simulink model "PSO_BON"  (R2019b)
settings: Solver=VariableStepAuto  StartTime=0.0  StopTime=0.2  RelTol=1e-5
undefined symbols (not defined in the file): sigbuilder_block
libraries: powerlib x164, re_lib x96, powerlib_meascontrol x9
(part 1 of 6)
settings Model: Creator=Mahesh Krishna  LastModifiedBy=nanaud
settings SolverCC: MaxConsecutiveZCs=1000000  AlgebraicLoopSolver=LineSearch  AutoInsertRateTranBlk=on
settings DataIOCC: ReturnWorkspaceOutputs=off
settings OptimizationCC: LifeSpan=inf
settings DebuggingCC: IgnoredZcDiagnostic=none  ArithmeticOperatorsInVariantConditions=warning
settings SFSimCC: SimUseLocalCustomCode=off  CustomCodeUndefinedFunction=UseInterfaceOnly
settings RTWCC: RTWUseLocalCustomCode=off
settings CodeAppCC: StateflowObjectComments=on
settings SimscapeCC: SimscapeNormalizeSystem=off

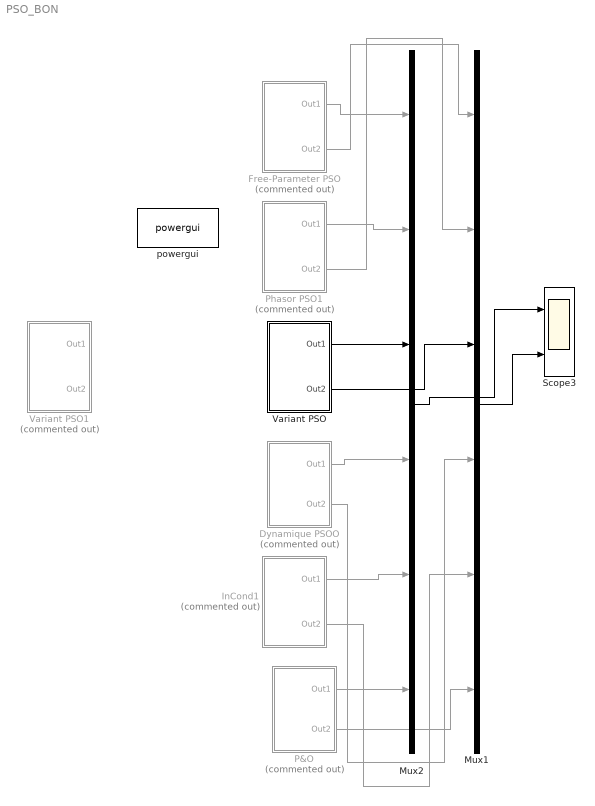
== system PSO_BON ==
  Dynamique PSOO : Subsystem  Commented=on
  Free-Parameter PSO : Subsystem  Commented=on
  InCond1 : Subsystem  Commented=on
  Mux1 : Mux  Inputs=6
  Mux2 : Mux  Inputs=6
  P&O : Subsystem  Commented=on
  Phasor PSO1 : Subsystem  Commented=on
  Scope3 : Scope  NumInputPorts=2
  Variant PSO : Subsystem
  Variant PSO1 : Subsystem  Commented=on
  powergui : powerlib/powergui  Priority=1  SimulationMode=Continuous  SampleTime=1e-6  frequency=60  Iterations=50  frequencyindice=0  Pbase=100e6  ErrMax=1e-4  UnitsV=kV  UnitsW=MW  buscounter=0  FunctionMessages=off  echomessages=off  EnableUseOfTLC=off  CurrentSourceSwitches=off  DisableSnubberDevices=off  DisableRonSwitches=off  DisableVfSwitches=off  DisplayEquations=off  AutomaticDiscreteSolvers=off  SolverType=Tustin/Backward Euler (TBE)  Interpol=off  ExternalGateDelay=off  methode=off  Ts=100  x0status=blocks  SPID=on  SwTol=0  HookPort=off  NonlinearTolerance=1e-4  nMaxIteration=100  ContinueOnMaxIteration=off  RestoreLinks=warning  ResistiveCurrentMeasurement=off  Frange=[0:2:500]  Ylog=off  Xlog=on  ShowGrid=off  save=off  variable=ZData  structure=0  ZoomFFT=off  StartTime=0.0  cycles=1  DisplayStyle=1  fundamental=60  FreqAxis=off  MaxFrequency=1000  frequencyindicesteady=1  RmsSteady=1  display=off
      settings: SourceProductName=Simscape Electrical
  wires:
  Mux2/1 -> Scope3/1
  Mux1/1 -> Scope3/2
  Free-Parameter PSO/1(Out1) -> Mux2/1
  P&O/1(Out1) -> Mux2/6
  InCond1/1(Out1) -> Mux2/5
  Dynamique PSOO/1(Out1) -> Mux2/4
  Variant PSO/1(Out1) -> Mux2/3
  Phasor PSO1/1(Out1) -> Mux2/2
  Free-Parameter PSO/2(Out2) -> Mux1/1
  Phasor PSO1/2(Out2) -> Mux1/2
  Variant PSO/2(Out2) -> Mux1/3
  Dynamique PSOO/2(Out2) -> Mux1/4
  InCond1/2(Out2) -> Mux1/5
  P&O/2(Out2) -> Mux1/6

== system PSO_BON/Dynamique PSOO ==
  Diode1 : powerlib/Power Electronics/Diode  Ron=1e-3  Lon=0  Vf=0  IC=0  UseSnubber=off  Rs=inf  Cs=inf  Measurements=off
      settings: SourceProductName=Simscape Electrical
  I : powerlib/Measurements/Current Measurement  PhasorSimulation=off  OutputType=Magnitude  PSBequivalent=0
      settings: SourceProductName=Simscape Electrical
  L : powerlib/Elements/Series RLC Branch  LConnTagsString=__new0  RConnTagsString=__new0  BranchType=L  Resistance=1e-3  Inductance=5e-3  SetiL0=off  InitialCurrent=0  Capacitance=1e-6  Setx0=off  InitialVoltage=0  Measurements=None
      settings: SourceProductName=Simscape Electrical
  M : powerlib/Power Electronics/Mosfet  Ron=1e-3  Lon=0  Rd=1e-3  Vfd=0  IC=0  Rs=inf  Cs=inf  Measurements=off
      settings: SourceProductName=Simscape Electrical
  MATLAB Function1 : MATLAB Function  TreatAsAtomicUnit=on
  Memory1 : Memory  LinearizeMemory=on
  Memory2 : Memory  LinearizeMemory=on
  Memory3 : Memory  LinearizeMemory=on
  PWM Generator (DC-DC)1 : powerlib_meascontrol/Pulse & Signal Generators/PWM Generator (DC-DC)  Fsw=40000  Ts=0
      settings: SourceProductName=Simscape Electrical
  Panel Surya : Subsystem
  Product1 : Product
  Saturation [0...1] : Saturate  UpperLimit=1  LowerLimit=0
  Series RLC Branch1 : powerlib/Elements/Series RLC Branch  LConnTagsString=__new0  RConnTagsString=__new0  BranchType=C  Resistance=1e-4  Inductance=200e-6  SetiL0=off  InitialCurrent=0  Capacitance=1e-6  Setx0=off  InitialVoltage=40  Measurements=None
      settings: SourceProductName=Simscape Electrical
  Series RLC Branch3 : powerlib/Elements/Series RLC Branch  LConnTagsString=__new0  RConnTagsString=__new0  BranchType=R  Resistance=100  Inductance=200e-6  SetiL0=off  InitialCurrent=0  Capacitance=1000e-6  Setx0=off  InitialVoltage=40  Measurements=None
      settings: SourceProductName=Simscape Electrical
  To Workspace4 : ToWorkspace  VariableName=Power5  SaveFormat=Structure With Time  SampleTime=-1
  To Workspace5 : ToWorkspace  VariableName=Duty5  SaveFormat=Structure With Time  SampleTime=-1
  Voltage Measurement1 : powerlib/Measurements/Voltage Measurement  PhasorSimulation=off  OutputType=Magnitude  PSBequivalent=0
      settings: SourceProductName=Simscape Electrical
  c : powerlib/Elements/Series RLC Branch  LConnTagsString=__new0  RConnTagsString=__new0  BranchType=C  Resistance=1e-3  Inductance=250e-6  SetiL0=off  InitialCurrent=0  Capacitance=10e-6  Setx0=off  InitialVoltage=0  Measurements=None
      settings: SourceProductName=Simscape Electrical
  Out1 : Outport
  Out2 : Outport  Port=2
  wires:
  Memory3/1 -> MATLAB Function1/2(Ipv)
  Memory2/1 -> MATLAB Function1/1(Vpv)
  I/1 -> [Ipv]
  Voltage Measurement1/1 -> [Vpv]
  PWM Generator (DC-DC)1/1 -> M/1
  Memory1/1 -> PWM Generator (DC-DC)1/1, To Workspace5/1, Out2/1
  Product1/1 -> To Workspace4/1, Out1/1
  [Ipv] -> Product1/1, Memory3/1
  [Vpv] -> Product1/2, Memory2/1
  MATLAB Function1/1(D) -> Saturation [0...1]/1
  Saturation [0...1]/1 -> Memory1/1
  connections:
  Panel Surya/RConn1 -- I/LConn1
  L/RConn1 -- M/LConn1 -- Diode1/LConn1
  Series RLC Branch1/LConn1 -- Diode1/RConn1 -- Series RLC Branch3/LConn1
  M/RConn1 -- Series RLC Branch3/RConn1 -- Series RLC Branch1/RConn1 -- c/RConn1 -- Panel Surya/RConn2 -- Voltage Measurement1/LConn2
  L/LConn1 -- c/LConn1 -- Voltage Measurement1/LConn1 -- I/RConn1

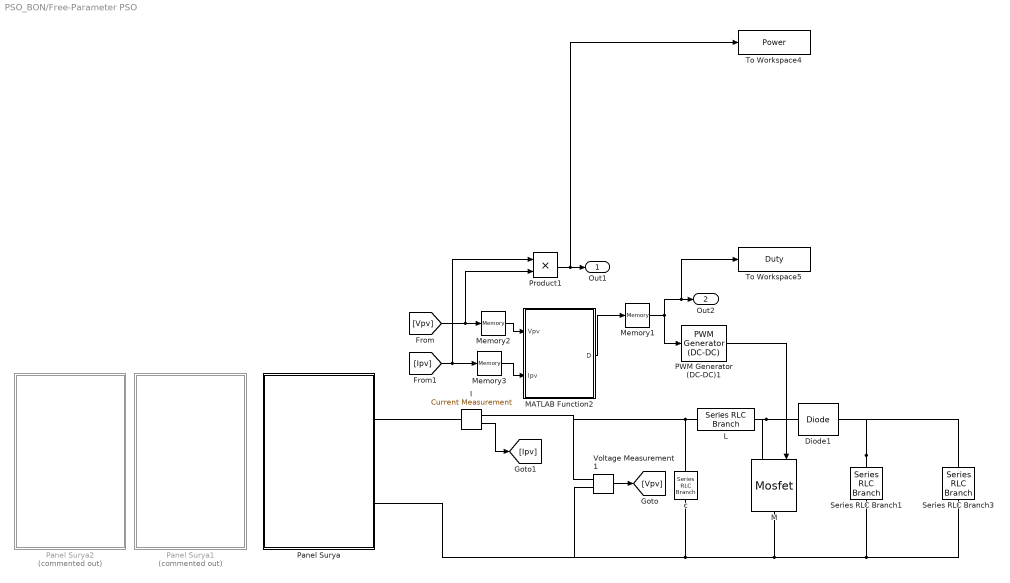
== system PSO_BON/Free-Parameter PSO ==
  Diode1 : powerlib/Power Electronics/Diode  Ron=1e-3  Lon=0  Vf=0  IC=0  UseSnubber=off  Rs=inf  Cs=inf  Measurements=off
      settings: SourceProductName=Simscape Electrical
  I : powerlib/Measurements/Current Measurement  PhasorSimulation=off  OutputType=Magnitude  PSBequivalent=0
      settings: SourceProductName=Simscape Electrical
  L : powerlib/Elements/Series RLC Branch  LConnTagsString=__new0  RConnTagsString=__new0  BranchType=L  Resistance=1e-3  Inductance=5e-3  SetiL0=off  InitialCurrent=0  Capacitance=1e-6  Setx0=off  InitialVoltage=0  Measurements=None
      settings: SourceProductName=Simscape Electrical
  M : powerlib/Power Electronics/Mosfet  Ron=1e-3  Lon=0  Rd=1e-3  Vfd=0  IC=0  Rs=inf  Cs=inf  Measurements=off
      settings: SourceProductName=Simscape Electrical
  MATLAB Function2 : MATLAB Function  TreatAsAtomicUnit=on
  Memory1 : Memory  LinearizeMemory=on
  Memory2 : Memory  LinearizeMemory=on
  Memory3 : Memory  LinearizeMemory=on
  PWM Generator (DC-DC)1 : powerlib_meascontrol/Pulse & Signal Generators/PWM Generator (DC-DC)  Fsw=40000  Ts=0
      settings: SourceProductName=Simscape Electrical
  Panel Surya : Subsystem
  Panel Surya1 : Subsystem  Commented=on
  Panel Surya2 : Subsystem  Commented=on
  Product1 : Product
  Series RLC Branch1 : powerlib/Elements/Series RLC Branch  LConnTagsString=__new0  RConnTagsString=__new0  BranchType=C  Resistance=1e-4  Inductance=200e-6  SetiL0=off  InitialCurrent=0  Capacitance=1e-6  Setx0=off  InitialVoltage=40  Measurements=None
      settings: SourceProductName=Simscape Electrical
  Series RLC Branch3 : powerlib/Elements/Series RLC Branch  LConnTagsString=__new0  RConnTagsString=__new0  BranchType=R  Resistance=100  Inductance=200e-6  SetiL0=off  InitialCurrent=0  Capacitance=1000e-6  Setx0=off  InitialVoltage=40  Measurements=None
      settings: SourceProductName=Simscape Electrical
  To Workspace4 : ToWorkspace  VariableName=Power  SaveFormat=Structure With Time  SampleTime=-1
  To Workspace5 : ToWorkspace  VariableName=Duty  SaveFormat=Structure With Time  SampleTime=-1
  Voltage Measurement1 : powerlib/Measurements/Voltage Measurement  PhasorSimulation=off  OutputType=Magnitude  PSBequivalent=0
      settings: SourceProductName=Simscape Electrical
  c : powerlib/Elements/Series RLC Branch  LConnTagsString=__new0  RConnTagsString=__new0  BranchType=C  Resistance=1e-3  Inductance=250e-6  SetiL0=off  InitialCurrent=0  Capacitance=10e-6  Setx0=off  InitialVoltage=0  Measurements=None
      settings: SourceProductName=Simscape Electrical
  Out1 : Outport
  Out2 : Outport  Port=2
  wires:
  Memory3/1 -> MATLAB Function2/2(Ipv)
  Memory2/1 -> MATLAB Function2/1(Vpv)
  I/1 -> [Ipv]
  Voltage Measurement1/1 -> [Vpv]
  PWM Generator (DC-DC)1/1 -> M/1
  Memory1/1 -> PWM Generator (DC-DC)1/1, To Workspace5/1, Out2/1
  Product1/1 -> To Workspace4/1, Out1/1
  [Ipv] -> Product1/1, Memory3/1
  MATLAB Function2/1(D) -> Memory1/1
  [Vpv] -> Product1/2, Memory2/1
  connections:
  Panel Surya/RConn1 -- I/LConn1
  L/RConn1 -- M/LConn1 -- Diode1/LConn1
  Series RLC Branch1/LConn1 -- Diode1/RConn1 -- Series RLC Branch3/LConn1
  M/RConn1 -- Series RLC Branch3/RConn1 -- Series RLC Branch1/RConn1 -- c/RConn1 -- Panel Surya/RConn2 -- Voltage Measurement1/LConn2
  L/LConn1 -- c/LConn1 -- Voltage Measurement1/LConn1 -- I/RConn1

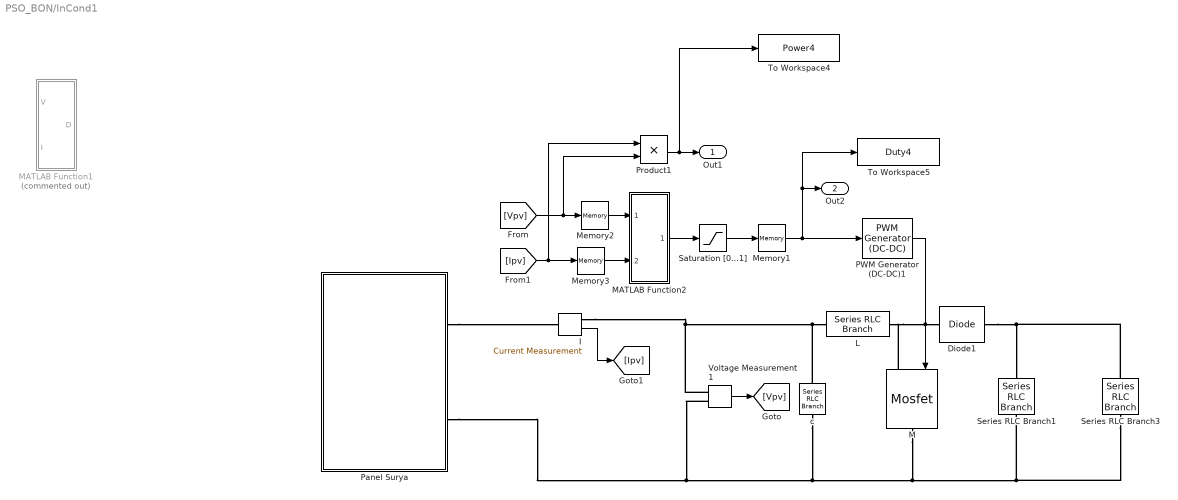
== system PSO_BON/InCond1 ==
  Diode1 : powerlib/Power Electronics/Diode  Ron=1e-3  Lon=0  Vf=0  IC=0  UseSnubber=off  Rs=inf  Cs=inf  Measurements=off
      settings: SourceProductName=Simscape Electrical
  I : powerlib/Measurements/Current Measurement  PhasorSimulation=off  OutputType=Magnitude  PSBequivalent=0
      settings: SourceProductName=Simscape Electrical
  L : powerlib/Elements/Series RLC Branch  LConnTagsString=__new0  RConnTagsString=__new0  BranchType=L  Resistance=1e-3  Inductance=5e-3  SetiL0=off  InitialCurrent=0  Capacitance=1e-6  Setx0=off  InitialVoltage=0  Measurements=None
      settings: SourceProductName=Simscape Electrical
  M : powerlib/Power Electronics/Mosfet  Ron=1e-3  Lon=0  Rd=1e-3  Vfd=0  IC=0  Rs=inf  Cs=inf  Measurements=off
      settings: SourceProductName=Simscape Electrical
  MATLAB Function1 : MATLAB Function  Commented=on  TreatAsAtomicUnit=on
  MATLAB Function2 : MATLAB Function  TreatAsAtomicUnit=on
  Memory1 : Memory  LinearizeMemory=on
  Memory2 : Memory  LinearizeMemory=on
  Memory3 : Memory  LinearizeMemory=on
  PWM Generator (DC-DC)1 : powerlib_meascontrol/Pulse & Signal Generators/PWM Generator (DC-DC)  Fsw=40000  Ts=0
      settings: SourceProductName=Simscape Electrical
  Panel Surya : Subsystem
  Product1 : Product
  Saturation [0...1] : Saturate  UpperLimit=1  LowerLimit=0
  Series RLC Branch1 : powerlib/Elements/Series RLC Branch  LConnTagsString=__new0  RConnTagsString=__new0  BranchType=C  Resistance=1e-4  Inductance=200e-6  SetiL0=off  InitialCurrent=0  Capacitance=1e-6  Setx0=off  InitialVoltage=40  Measurements=None
      settings: SourceProductName=Simscape Electrical
  Series RLC Branch3 : powerlib/Elements/Series RLC Branch  LConnTagsString=__new0  RConnTagsString=__new0  BranchType=R  Resistance=100  Inductance=200e-6  SetiL0=off  InitialCurrent=0  Capacitance=1000e-6  Setx0=off  InitialVoltage=40  Measurements=None
      settings: SourceProductName=Simscape Electrical
  To Workspace4 : ToWorkspace  VariableName=Power4  SaveFormat=Structure With Time  SampleTime=-1
  To Workspace5 : ToWorkspace  VariableName=Duty4  SaveFormat=Structure With Time  SampleTime=-1
  Voltage Measurement1 : powerlib/Measurements/Voltage Measurement  PhasorSimulation=off  OutputType=Magnitude  PSBequivalent=0
      settings: SourceProductName=Simscape Electrical
  c : powerlib/Elements/Series RLC Branch  LConnTagsString=__new0  RConnTagsString=__new0  BranchType=C  Resistance=1e-3  Inductance=250e-6  SetiL0=off  InitialCurrent=0  Capacitance=10e-6  Setx0=off  InitialVoltage=0  Measurements=None
      settings: SourceProductName=Simscape Electrical
  Out1 : Outport
  Out2 : Outport  Port=2
  wires:
  Saturation [0...1]/1 -> Memory1/1
  MATLAB Function2/1(Duty) -> Saturation [0...1]/1
  [Vpv] -> Memory2/1, Product1/2
  [Ipv] -> Memory3/1, Product1/1
  Product1/1 -> Out1/1, To Workspace4/1
  Memory1/1 -> Out2/1, To Workspace5/1, PWM Generator (DC-DC)1/1
  PWM Generator (DC-DC)1/1 -> M/1
  Voltage Measurement1/1 -> [Vpv]
  I/1 -> [Ipv]
  Memory2/1 -> MATLAB Function2/1(Vpv)
  Memory3/1 -> MATLAB Function2/2(Ipv)
  connections:
  I/RConn1 -- Voltage Measurement1/LConn1 -- c/LConn1 -- L/LConn1
  Voltage Measurement1/LConn2 -- Panel Surya/RConn2 -- c/RConn1 -- Series RLC Branch1/RConn1 -- Series RLC Branch3/RConn1 -- M/RConn1
  Series RLC Branch3/LConn1 -- Diode1/RConn1 -- Series RLC Branch1/LConn1
  Diode1/LConn1 -- M/LConn1 -- L/RConn1
  Panel Surya/RConn1 -- I/LConn1

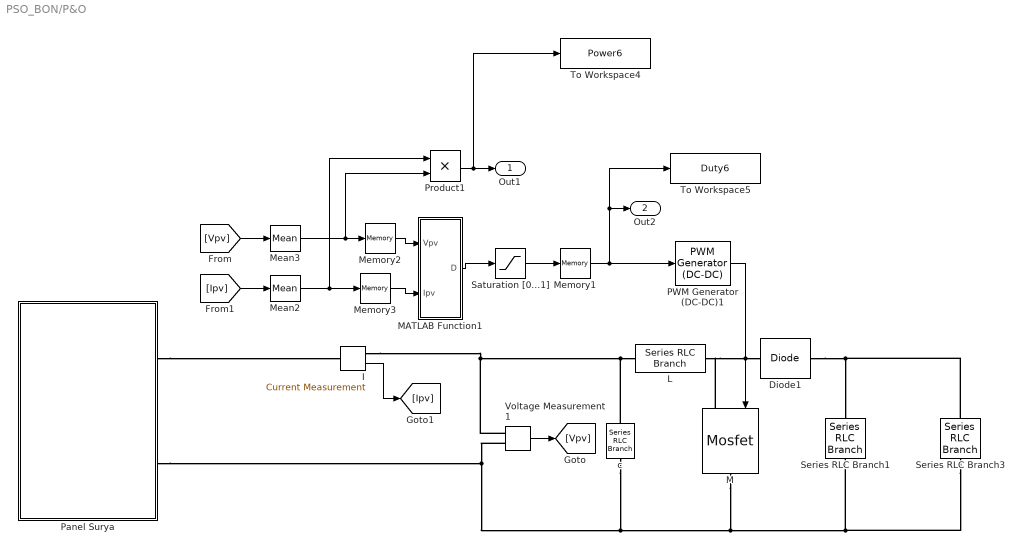
== system PSO_BON/P&O ==
  Diode1 : powerlib/Power Electronics/Diode  Ron=1e-3  Lon=0  Vf=0  IC=0  UseSnubber=off  Rs=inf  Cs=inf  Measurements=off
      settings: SourceProductName=Simscape Electrical
  I : powerlib/Measurements/Current Measurement  PhasorSimulation=off  OutputType=Magnitude  PSBequivalent=0
      settings: SourceProductName=Simscape Electrical
  L : powerlib/Elements/Series RLC Branch  LConnTagsString=__new0  RConnTagsString=__new0  BranchType=L  Resistance=1e-3  Inductance=5e-3  SetiL0=off  InitialCurrent=0  Capacitance=1e-6  Setx0=off  InitialVoltage=0  Measurements=None
      settings: SourceProductName=Simscape Electrical
  M : powerlib/Power Electronics/Mosfet  Ron=1e-3  Lon=0  Rd=1e-3  Vfd=0  IC=0  Rs=inf  Cs=inf  Measurements=off
      settings: SourceProductName=Simscape Electrical
  MATLAB Function1 : MATLAB Function  TreatAsAtomicUnit=on
  Mean2 : powerlib_meascontrol/Measurements/Mean  Freq=40000  Vinit=0  Ts=0
      settings: SourceProductName=Simscape Electrical
  Mean3 : powerlib_meascontrol/Measurements/Mean  Freq=40000  Vinit=0  Ts=0
      settings: SourceProductName=Simscape Electrical
  Memory1 : Memory  LinearizeMemory=on
  Memory2 : Memory  LinearizeMemory=on
  Memory3 : Memory  LinearizeMemory=on
  PWM Generator (DC-DC)1 : powerlib_meascontrol/Pulse & Signal Generators/PWM Generator (DC-DC)  Fsw=40000  Ts=0
      settings: SourceProductName=Simscape Electrical
  Panel Surya : Subsystem
  Product1 : Product
  Saturation [0...1] : Saturate  UpperLimit=1  LowerLimit=0
  Series RLC Branch1 : powerlib/Elements/Series RLC Branch  LConnTagsString=__new0  RConnTagsString=__new0  BranchType=C  Resistance=1e-4  Inductance=200e-6  SetiL0=off  InitialCurrent=0  Capacitance=1e-6  Setx0=off  InitialVoltage=40  Measurements=None
      settings: SourceProductName=Simscape Electrical
  Series RLC Branch3 : powerlib/Elements/Series RLC Branch  LConnTagsString=__new0  RConnTagsString=__new0  BranchType=R  Resistance=100  Inductance=200e-6  SetiL0=off  InitialCurrent=0  Capacitance=1000e-6  Setx0=off  InitialVoltage=40  Measurements=None
      settings: SourceProductName=Simscape Electrical
  To Workspace4 : ToWorkspace  VariableName=Power6  SaveFormat=Structure With Time  SampleTime=-1
  To Workspace5 : ToWorkspace  VariableName=Duty6  SaveFormat=Structure With Time  SampleTime=-1
  Voltage Measurement1 : powerlib/Measurements/Voltage Measurement  PhasorSimulation=off  OutputType=Magnitude  PSBequivalent=0
      settings: SourceProductName=Simscape Electrical
  c : powerlib/Elements/Series RLC Branch  LConnTagsString=__new0  RConnTagsString=__new0  BranchType=C  Resistance=1e-3  Inductance=250e-6  SetiL0=off  InitialCurrent=0  Capacitance=10e-6  Setx0=off  InitialVoltage=0  Measurements=None
      settings: SourceProductName=Simscape Electrical
  Out1 : Outport
  Out2 : Outport  Port=2
  wires:
  Saturation [0...1]/1 -> Memory1/1
  MATLAB Function1/1(D) -> Saturation [0...1]/1
  [Vpv] -> Mean3/1
  [Ipv] -> Mean2/1
  Product1/1 -> Out1/1, To Workspace4/1
  Memory1/1 -> Out2/1, To Workspace5/1, PWM Generator (DC-DC)1/1
  PWM Generator (DC-DC)1/1 -> M/1
  Voltage Measurement1/1 -> [Vpv]
  I/1 -> [Ipv]
  Memory2/1 -> MATLAB Function1/1(Vpv)
  Memory3/1 -> MATLAB Function1/2(Ipv)
  Mean2/1 -> Memory3/1, Product1/1
  Mean3/1 -> Memory2/1, Product1/2
  connections:
  I/RConn1 -- Voltage Measurement1/LConn1 -- c/LConn1 -- L/LConn1
  Voltage Measurement1/LConn2 -- c/RConn1 -- Series RLC Branch1/RConn1 -- Series RLC Branch3/RConn1 -- M/RConn1 -- Panel Surya/RConn2
  Series RLC Branch3/LConn1 -- Diode1/RConn1 -- Series RLC Branch1/LConn1
  Diode1/LConn1 -- M/LConn1 -- L/RConn1
  Panel Surya/RConn1 -- I/LConn1

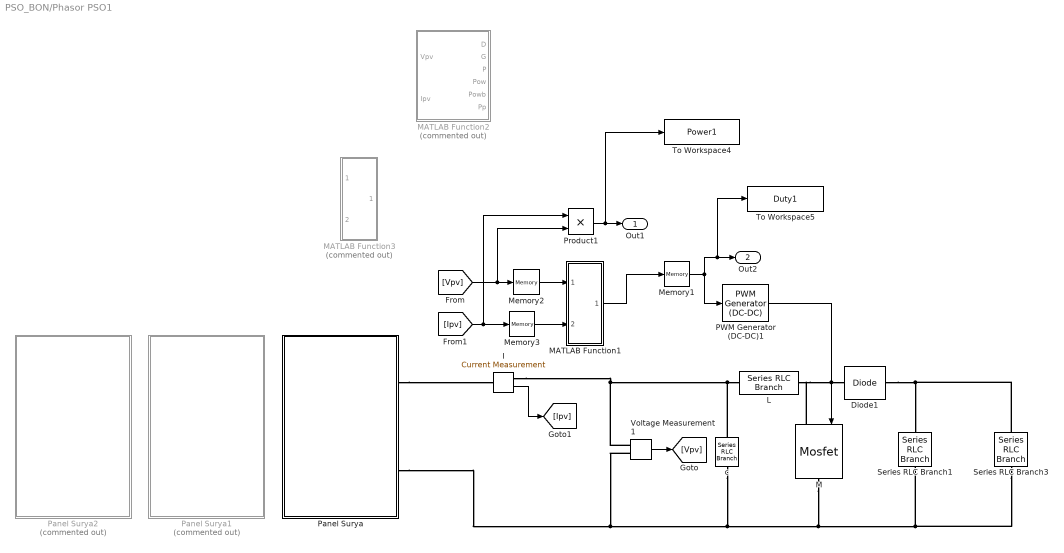
== system PSO_BON/Phasor PSO1 ==
  Diode1 : powerlib/Power Electronics/Diode  Ron=1e-3  Lon=0  Vf=0  IC=0  UseSnubber=off  Rs=inf  Cs=inf  Measurements=off
      settings: SourceProductName=Simscape Electrical
  I : powerlib/Measurements/Current Measurement  PhasorSimulation=off  OutputType=Magnitude  PSBequivalent=0
      settings: SourceProductName=Simscape Electrical
  L : powerlib/Elements/Series RLC Branch  LConnTagsString=__new0  RConnTagsString=__new0  BranchType=L  Resistance=1e-3  Inductance=5e-3  SetiL0=off  InitialCurrent=0  Capacitance=1e-6  Setx0=off  InitialVoltage=0  Measurements=None
      settings: SourceProductName=Simscape Electrical
  M : powerlib/Power Electronics/Mosfet  Ron=1e-3  Lon=0  Rd=1e-3  Vfd=0  IC=0  Rs=inf  Cs=inf  Measurements=off
      settings: SourceProductName=Simscape Electrical
  MATLAB Function1 : MATLAB Function  TreatAsAtomicUnit=on
  MATLAB Function2 : MATLAB Function  Commented=on  TreatAsAtomicUnit=on
  MATLAB Function3 : MATLAB Function  Commented=on  TreatAsAtomicUnit=on
  Memory1 : Memory  LinearizeMemory=on
  Memory2 : Memory  LinearizeMemory=on
  Memory3 : Memory  LinearizeMemory=on
  PWM Generator (DC-DC)1 : powerlib_meascontrol/Pulse & Signal Generators/PWM Generator (DC-DC)  Fsw=40000  Ts=0
      settings: SourceProductName=Simscape Electrical
  Panel Surya : Subsystem
  Panel Surya1 : Subsystem  Commented=on
  Panel Surya2 : Subsystem  Commented=on
  Product1 : Product
  Series RLC Branch1 : powerlib/Elements/Series RLC Branch  LConnTagsString=__new0  RConnTagsString=__new0  BranchType=C  Resistance=1e-4  Inductance=200e-6  SetiL0=off  InitialCurrent=0  Capacitance=1e-6  Setx0=off  InitialVoltage=40  Measurements=None
      settings: SourceProductName=Simscape Electrical
  Series RLC Branch3 : powerlib/Elements/Series RLC Branch  LConnTagsString=__new0  RConnTagsString=__new0  BranchType=R  Resistance=100  Inductance=200e-6  SetiL0=off  InitialCurrent=0  Capacitance=1000e-6  Setx0=off  InitialVoltage=40  Measurements=None
      settings: SourceProductName=Simscape Electrical
  To Workspace4 : ToWorkspace  VariableName=Power1  SaveFormat=Structure With Time  SampleTime=-1
  To Workspace5 : ToWorkspace  VariableName=Duty1  SaveFormat=Structure With Time  SampleTime=-1
  Voltage Measurement1 : powerlib/Measurements/Voltage Measurement  PhasorSimulation=off  OutputType=Magnitude  PSBequivalent=0
      settings: SourceProductName=Simscape Electrical
  c : powerlib/Elements/Series RLC Branch  LConnTagsString=__new0  RConnTagsString=__new0  BranchType=C  Resistance=1e-3  Inductance=250e-6  SetiL0=off  InitialCurrent=0  Capacitance=10e-6  Setx0=off  InitialVoltage=0  Measurements=None
      settings: SourceProductName=Simscape Electrical
  Out1 : Outport
  Out2 : Outport  Port=2
  wires:
  [Vpv] -> Memory2/1, Product1/2
  MATLAB Function1/1(Duty) -> Memory1/1
  [Ipv] -> Memory3/1, Product1/1
  Product1/1 -> To Workspace4/1, Out1/1
  Memory1/1 -> To Workspace5/1, Out2/1, PWM Generator (DC-DC)1/1
  PWM Generator (DC-DC)1/1 -> M/1
  Voltage Measurement1/1 -> [Vpv]
  I/1 -> [Ipv]
  Memory2/1 -> MATLAB Function1/1(Vpv)
  Memory3/1 -> MATLAB Function1/2(Ipv)
  connections:
  I/RConn1 -- Voltage Measurement1/LConn1 -- c/LConn1 -- L/LConn1
  Voltage Measurement1/LConn2 -- Panel Surya/RConn2 -- c/RConn1 -- Series RLC Branch1/RConn1 -- Series RLC Branch3/RConn1 -- M/RConn1
  Series RLC Branch3/LConn1 -- Diode1/RConn1 -- Series RLC Branch1/LConn1
  Diode1/LConn1 -- M/LConn1 -- L/RConn1
  Panel Surya/RConn1 -- I/LConn1

== system PSO_BON/Variant PSO ==
  Diode1 : powerlib/Power Electronics/Diode  Ron=1e-3  Lon=0  Vf=0  IC=0  UseSnubber=off  Rs=inf  Cs=inf  Measurements=off
      settings: SourceProductName=Simscape Electrical
  I : powerlib/Measurements/Current Measurement  PhasorSimulation=off  OutputType=Magnitude  PSBequivalent=0
      settings: SourceProductName=Simscape Electrical
  L : powerlib/Elements/Series RLC Branch  LConnTagsString=__new0  RConnTagsString=__new0  BranchType=L  Resistance=1e-3  Inductance=5e-3  SetiL0=off  InitialCurrent=0  Capacitance=1e-6  Setx0=off  InitialVoltage=0  Measurements=None
      settings: SourceProductName=Simscape Electrical
  M : powerlib/Power Electronics/Mosfet  Ron=1e-3  Lon=0  Rd=1e-3  Vfd=0  IC=0  Rs=inf  Cs=inf  Measurements=off
      settings: SourceProductName=Simscape Electrical
  MATLAB Function1 : MATLAB Function  TreatAsAtomicUnit=on
  Memory1 : Memory  LinearizeMemory=on
  Memory2 : Memory  LinearizeMemory=on
  Memory3 : Memory  LinearizeMemory=on
  PWM Generator (DC-DC)1 : powerlib_meascontrol/Pulse & Signal Generators/PWM Generator (DC-DC)  Fsw=40000  Ts=0
      settings: SourceProductName=Simscape Electrical
  Panel Surya : Subsystem
  Product1 : Product
  Saturation [0...1] : Saturate  UpperLimit=1  LowerLimit=0
  Series RLC Branch1 : powerlib/Elements/Series RLC Branch  LConnTagsString=__new0  RConnTagsString=__new0  BranchType=C  Resistance=1e-4  Inductance=200e-6  SetiL0=off  InitialCurrent=0  Capacitance=1e-6  Setx0=off  InitialVoltage=40  Measurements=None
      settings: SourceProductName=Simscape Electrical
  Series RLC Branch3 : powerlib/Elements/Series RLC Branch  LConnTagsString=__new0  RConnTagsString=__new0  BranchType=R  Resistance=100  Inductance=200e-6  SetiL0=off  InitialCurrent=0  Capacitance=1000e-6  Setx0=off  InitialVoltage=40  Measurements=None
      settings: SourceProductName=Simscape Electrical
  To Workspace4 : ToWorkspace  VariableName=Power3  SaveFormat=Structure With Time  SampleTime=-1
  To Workspace5 : ToWorkspace  VariableName=Duty3  SaveFormat=Structure With Time  SampleTime=-1
  Voltage Measurement1 : powerlib/Measurements/Voltage Measurement  PhasorSimulation=off  OutputType=Magnitude  PSBequivalent=0
      settings: SourceProductName=Simscape Electrical
  c : powerlib/Elements/Series RLC Branch  LConnTagsString=__new0  RConnTagsString=__new0  BranchType=C  Resistance=1e-3  Inductance=250e-6  SetiL0=off  InitialCurrent=0  Capacitance=10e-6  Setx0=off  InitialVoltage=0  Measurements=None
      settings: SourceProductName=Simscape Electrical
  Out1 : Outport
  Out2 : Outport  Port=2
  wires:
  Memory3/1 -> MATLAB Function1/2(Ipv)
  Memory2/1 -> MATLAB Function1/1(Vpv)
  I/1 -> [Ipv]
  Voltage Measurement1/1 -> [Vpv]
  PWM Generator (DC-DC)1/1 -> M/1
  Memory1/1 -> PWM Generator (DC-DC)1/1, To Workspace5/1, Out2/1
  Product1/1 -> To Workspace4/1, Out1/1
  [Ipv] -> Product1/1, Memory3/1
  [Vpv] -> Product1/2, Memory2/1
  MATLAB Function1/1(Duty) -> Saturation [0...1]/1
  Saturation [0...1]/1 -> Memory1/1
  connections:
  Panel Surya/RConn1 -- I/LConn1
  L/RConn1 -- M/LConn1 -- Diode1/LConn1
  Series RLC Branch1/LConn1 -- Diode1/RConn1 -- Series RLC Branch3/LConn1
  M/RConn1 -- Series RLC Branch3/RConn1 -- Series RLC Branch1/RConn1 -- Panel Surya/RConn2 -- Voltage Measurement1/LConn2 -- c/RConn1
  L/LConn1 -- c/LConn1 -- Voltage Measurement1/LConn1 -- I/RConn1

== system PSO_BON/Variant PSO1 ==
  Diode1 : powerlib/Power Electronics/Diode  Ron=1e-3  Lon=0  Vf=0  IC=0  UseSnubber=off  Rs=inf  Cs=inf  Measurements=off
      settings: SourceProductName=Simscape Electrical
  I : powerlib/Measurements/Current Measurement  PhasorSimulation=off  OutputType=Magnitude  PSBequivalent=0
      settings: SourceProductName=Simscape Electrical
  L : powerlib/Elements/Series RLC Branch  LConnTagsString=__new0  RConnTagsString=__new0  BranchType=L  Resistance=1e-3  Inductance=5e-3  SetiL0=off  InitialCurrent=0  Capacitance=1e-6  Setx0=off  InitialVoltage=0  Measurements=None
      settings: SourceProductName=Simscape Electrical
  M : powerlib/Power Electronics/Mosfet  Ron=1e-3  Lon=0  Rd=1e-3  Vfd=0  IC=0  Rs=inf  Cs=inf  Measurements=off
      settings: SourceProductName=Simscape Electrical
  MATLAB Function1 : MATLAB Function  TreatAsAtomicUnit=on
  Memory1 : Memory  LinearizeMemory=on
  Memory2 : Memory  LinearizeMemory=on
  Memory3 : Memory  LinearizeMemory=on
  PWM Generator (DC-DC)1 : powerlib_meascontrol/Pulse & Signal Generators/PWM Generator (DC-DC)  Fsw=40000  Ts=0
      settings: SourceProductName=Simscape Electrical
  Panel Surya : Subsystem
  Product1 : Product
  Saturation [0...1] : Saturate  UpperLimit=1  LowerLimit=0
  Series RLC Branch1 : powerlib/Elements/Series RLC Branch  LConnTagsString=__new0  RConnTagsString=__new0  BranchType=C  Resistance=1e-4  Inductance=200e-6  SetiL0=off  InitialCurrent=0  Capacitance=1e-6  Setx0=off  InitialVoltage=40  Measurements=None
      settings: SourceProductName=Simscape Electrical
  Series RLC Branch3 : powerlib/Elements/Series RLC Branch  LConnTagsString=__new0  RConnTagsString=__new0  BranchType=R  Resistance=100  Inductance=200e-6  SetiL0=off  InitialCurrent=0  Capacitance=1000e-6  Setx0=off  InitialVoltage=40  Measurements=None
      settings: SourceProductName=Simscape Electrical
  To Workspace4 : ToWorkspace  VariableName=Power3  SaveFormat=Structure With Time  SampleTime=-1
  To Workspace5 : ToWorkspace  VariableName=Duty3  SaveFormat=Structure With Time  SampleTime=-1
  Voltage Measurement1 : powerlib/Measurements/Voltage Measurement  PhasorSimulation=off  OutputType=Magnitude  PSBequivalent=0
      settings: SourceProductName=Simscape Electrical
  c : powerlib/Elements/Series RLC Branch  LConnTagsString=__new0  RConnTagsString=__new0  BranchType=C  Resistance=1e-3  Inductance=250e-6  SetiL0=off  InitialCurrent=0  Capacitance=10e-6  Setx0=off  InitialVoltage=0  Measurements=None
      settings: SourceProductName=Simscape Electrical
  Out1 : Outport
  Out2 : Outport  Port=2
  wires:
  Saturation [0...1]/1 -> Memory1/1
  MATLAB Function1/1(D) -> Saturation [0...1]/1
  [Vpv] -> Memory2/1, Product1/2
  [Ipv] -> Memory3/1, Product1/1
  Product1/1 -> Out1/1, To Workspace4/1
  Memory1/1 -> Out2/1, To Workspace5/1, PWM Generator (DC-DC)1/1
  PWM Generator (DC-DC)1/1 -> M/1
  Voltage Measurement1/1 -> [Vpv]
  I/1 -> [Ipv]
  Memory2/1 -> MATLAB Function1/1(Vpv)
  Memory3/1 -> MATLAB Function1/2(Ipv)
  connections:
  I/RConn1 -- Voltage Measurement1/LConn1 -- c/LConn1 -- L/LConn1
  c/RConn1 -- Voltage Measurement1/LConn2 -- Panel Surya/RConn2 -- Series RLC Branch1/RConn1 -- Series RLC Branch3/RConn1 -- M/RConn1
  Series RLC Branch3/LConn1 -- Diode1/RConn1 -- Series RLC Branch1/LConn1
  Diode1/LConn1 -- M/LConn1 -- L/RConn1
  Panel Surya/RConn1 -- I/LConn1

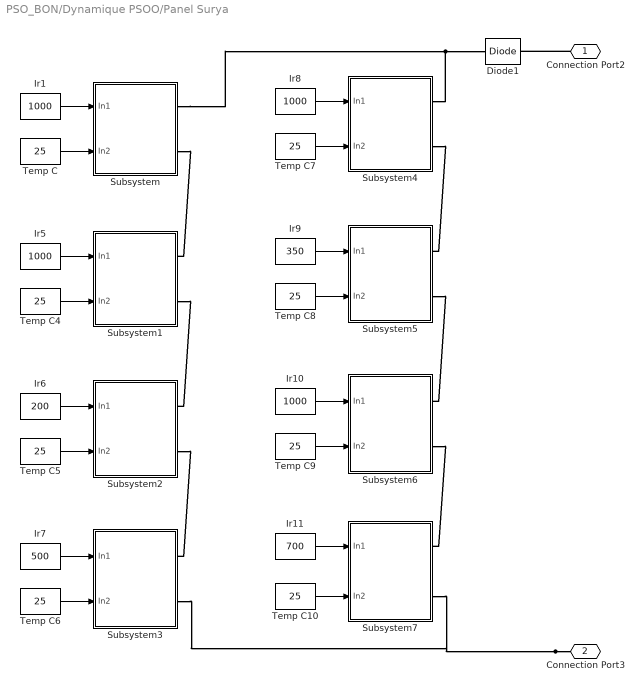
== system PSO_BON/Dynamique PSOO/Panel Surya ==
  Diode1 : powerlib/Power Electronics/Diode  Ron=0.001  Lon=0  Vf=0.7  IC=0  UseSnubber=off  Rs=1e5*inf  Cs=inf  Measurements=off
      settings: SourceProductName=Simscape Electrical
  Ir{1,5,8,10} (4 alike) : Constant  Value=1000
  Ir11 : Constant  Value=700
  Ir6 : Constant  Value=200
  Ir7 : Constant  Value=500
  Ir9 : Constant  Value=350
  Subsystem : Subsystem
  Subsystem1 : Subsystem
  Subsystem2 : Subsystem
  Subsystem3 : Subsystem
  Subsystem4 : Subsystem
  Subsystem5 : Subsystem
  Subsystem6 : Subsystem
  Subsystem7 : Subsystem
  Temp C{,4..10} (8 alike) : Constant  Value=25
  Connection Port2 : PMIOPort  Side=Right
  Connection Port3 : PMIOPort  Port=2  Side=Right
  wires:
  Temp C10/1 -> Subsystem7/2(In2)
  Ir10/1 -> Subsystem6/1(In1)
  Temp C9/1 -> Subsystem6/2(In2)
  Ir9/1 -> Subsystem5/1(In1)
  Ir11/1 -> Subsystem7/1(In1)
  Temp C8/1 -> Subsystem5/2(In2)
  Temp C7/1 -> Subsystem4/2(In2)
  Ir8/1 -> Subsystem4/1(In1)
  Ir6/1 -> Subsystem2/1(In1)
  Ir5/1 -> Subsystem1/1(In1)
  Temp C4/1 -> Subsystem1/2(In2)
  Temp C5/1 -> Subsystem2/2(In2)
  Temp C/1 -> Subsystem/2(In2)
  Ir1/1 -> Subsystem/1(In1)
  Temp C6/1 -> Subsystem3/2(In2)
  Ir7/1 -> Subsystem3/1(In1)
  connections:
  Connection Port2/RConn1 -- Diode1/RConn1
  Subsystem5/RConn2 -- Subsystem6/RConn1
  Subsystem6/RConn2 -- Subsystem7/RConn1
  Subsystem1/RConn2 -- Subsystem2/RConn1
  Subsystem2/RConn2 -- Subsystem3/RConn1
  Subsystem/RConn2 -- Subsystem1/RConn1
  Subsystem4/RConn2 -- Subsystem5/RConn1
  Subsystem/RConn1 -- Subsystem4/RConn1 -- Diode1/LConn1
  Connection Port3/RConn1 -- Subsystem7/RConn2 -- Subsystem3/RConn2

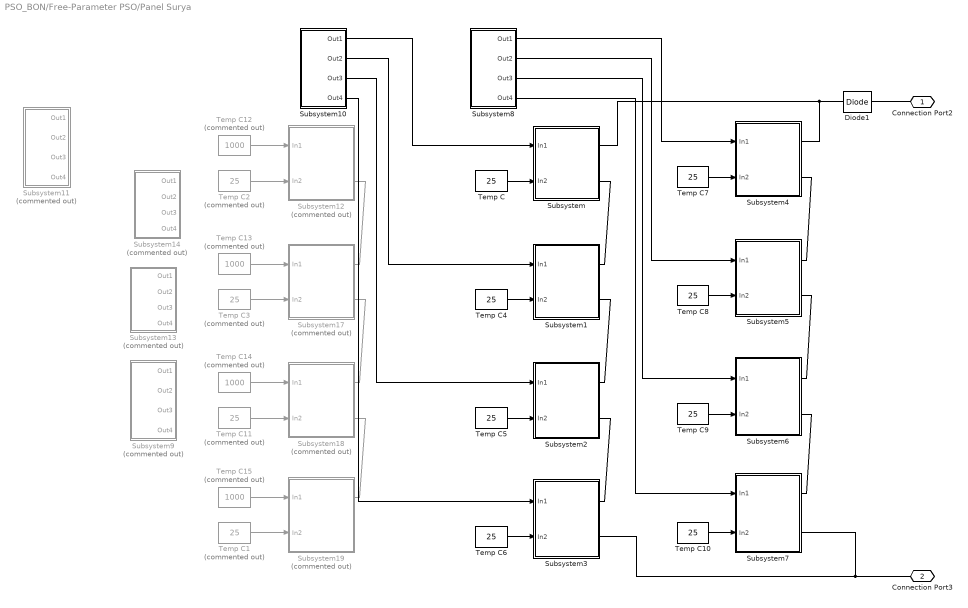
== system PSO_BON/Free-Parameter PSO/Panel Surya ==
  Diode1 : powerlib/Power Electronics/Diode  Ron=0.001  Lon=0  Vf=0.7  IC=0  UseSnubber=off  Rs=1e5*inf  Cs=inf  Measurements=off
      settings: SourceProductName=Simscape Electrical
  Subsystem : Subsystem
  Subsystem1 : Subsystem
  Subsystem10 : Subsystem
  Subsystem11 : Subsystem  Commented=on
  Subsystem12 : Subsystem  Commented=on
  Subsystem13 : Subsystem  Commented=on
  Subsystem14 : Subsystem  Commented=on
  Subsystem17 : Subsystem  Commented=on
  Subsystem18 : Subsystem  Commented=on
  Subsystem19 : Subsystem  Commented=on
  Subsystem2 : Subsystem
  Subsystem3 : Subsystem
  Subsystem4 : Subsystem
  Subsystem5 : Subsystem
  Subsystem6 : Subsystem
  Subsystem7 : Subsystem
  Subsystem8 : Subsystem
  Subsystem9 : Subsystem  Commented=on
  Temp C{,4..10} (8 alike) : Constant  Value=25
  Temp C{1..3,11} (4 alike) : Constant  Commented=on  Value=25
  Temp C{12..15} (4 alike) : Constant  Commented=on  Value=1000
  Connection Port2 : PMIOPort  Side=Right
  Connection Port3 : PMIOPort  Port=2  Side=Right
  wires:
  Temp C10/1 -> Subsystem7/2(In2)
  Temp C9/1 -> Subsystem6/2(In2)
  Temp C8/1 -> Subsystem5/2(In2)
  Temp C7/1 -> Subsystem4/2(In2)
  Temp C4/1 -> Subsystem1/2(In2)
  Temp C5/1 -> Subsystem2/2(In2)
  Temp C/1 -> Subsystem/2(In2)
  Temp C6/1 -> Subsystem3/2(In2)
  Subsystem8/2(Out2) -> Subsystem5/1(In1)
  Subsystem8/3(Out3) -> Subsystem6/1(In1)
  Subsystem8/1(Out1) -> Subsystem4/1(In1)
  Subsystem8/4(Out4) -> Subsystem7/1(In1)
  Temp C12/1 -> Subsystem12/1(In1)
  Temp C2/1 -> Subsystem12/2(In2)
  Temp C13/1 -> Subsystem17/1(In1)
  Temp C3/1 -> Subsystem17/2(In2)
  Temp C14/1 -> Subsystem18/1(In1)
  Temp C11/1 -> Subsystem18/2(In2)
  Temp C15/1 -> Subsystem19/1(In1)
  Temp C1/1 -> Subsystem19/2(In2)
  Subsystem10/1(Out1) -> Subsystem/1(In1)
  Subsystem10/2(Out2) -> Subsystem1/1(In1)
  Subsystem10/3(Out3) -> Subsystem2/1(In1)
  Subsystem10/4(Out4) -> Subsystem3/1(In1)
  connections:
  Connection Port2/RConn1 -- Diode1/RConn1
  Subsystem5/RConn2 -- Subsystem6/RConn1
  Subsystem6/RConn2 -- Subsystem7/RConn1
  Subsystem1/RConn2 -- Subsystem2/RConn1
  Subsystem2/RConn2 -- Subsystem3/RConn1
  Subsystem/RConn2 -- Subsystem1/RConn1
  Subsystem4/RConn2 -- Subsystem5/RConn1
  Subsystem12/RConn2 -- Subsystem17/RConn1
  Subsystem17/RConn2 -- Subsystem18/RConn1
  Subsystem18/RConn2 -- Subsystem19/RConn1
  Subsystem7/RConn2 -- Subsystem3/RConn2 -- Connection Port3/RConn1
  Subsystem/RConn1 -- Subsystem4/RConn1 -- Diode1/LConn1

== system PSO_BON/Free-Parameter PSO/Panel Surya1 ==
  Bypass Diode {5..8} (4 alike) : powerlib/Power Electronics/Diode  Ron=0.001  Lon=0  Vf=0.8  IC=0  UseSnubber=off  Rs=500  Cs=250e-9  Measurements=off
      settings: SourceProductName=Simscape Electrical
  Demux2 : Demux
  Demux3 : Demux
  Intensitas Radiasi1 : Constant  Value=[1000 700 100 200]
  PV Module 1 : re_lib/Solar/PV Array  Npar=2  Nser=1  PlotType=array @ 1000 W/m2 & specified temperatures  S_vec="[ 1000  500  100 ]"  Temp_C_vec="[ 45 25  ]"  ModuleName=SunPower SPR-315E-WHT-D  PlotWhenSelected=off  Pm=315.072  Ncell=96  Voc=64.6  Isc=6.14  Vm=54.7  Im=5.76  beta_Voc_pc=-0.27269  alpha_Isc_pc=0.061694  beta_Voc=-0.17616  alpha_Isc=0.003788  IL=6.1461  I0=6.5043e-12  nI=0.9507  Rsh=430.0559  Rs=0.43042  BAL=off  Tc=1e-6  Tfilter=5e-5
      settings: SourceProductName=Simscape Electrical
  PV Module 2 : re_lib/Solar/PV Array  Npar=2  Nser=1  PlotType=array @ 1000 W/m2 & specified temperatures  S_vec="[ 1000  500  100 ]"  Temp_C_vec="[ 45 25  ]"  ModuleName=SunPower SPR-315E-WHT-D  PlotWhenSelected=off  Pm=315.072  Ncell=96  Voc=64.6  Isc=6.14  Vm=54.7  Im=5.76  beta_Voc_pc=-0.27269  alpha_Isc_pc=0.061694  beta_Voc=-0.17616  alpha_Isc=0.003788  IL=6.1461  I0=6.5043e-12  nI=0.9507  Rsh=430.0559  Rs=0.43042  BAL=off  Tc=1e-6  Tfilter=5e-5
      settings: SourceProductName=Simscape Electrical
  PV Module 3 : re_lib/Solar/PV Array  Npar=2  Nser=1  PlotType=array @ 1000 W/m2 & specified temperatures  S_vec="[ 1000  500  100 ]"  Temp_C_vec="[ 45 25  ]"  ModuleName=SunPower SPR-315E-WHT-D  PlotWhenSelected=off  Pm=315.072  Ncell=96  Voc=64.6  Isc=6.14  Vm=54.7  Im=5.76  beta_Voc_pc=-0.27269  alpha_Isc_pc=0.061694  beta_Voc=-0.17616  alpha_Isc=0.003788  IL=6.1461  I0=6.5043e-12  nI=0.9507  Rsh=430.0559  Rs=0.43042  BAL=off  Tc=1e-6  Tfilter=5e-5
      settings: SourceProductName=Simscape Electrical
  PV Module 5 : re_lib/Solar/PV Array  Npar=2  Nser=1  PlotType=one module @ 25 deg.C & specified irradiances  S_vec="[ 1000  800  100 200]"  Temp_C_vec="[ 45 25  ]"  ModuleName=SunPower SPR-315E-WHT-D  PlotWhenSelected=off  Pm=315.072  Ncell=96  Voc=64.6  Isc=6.14  Vm=54.7  Im=5.76  beta_Voc_pc=-0.27269  alpha_Isc_pc=0.061694  beta_Voc=-0.17616  alpha_Isc=0.003788  IL=6.1461  I0=6.5043e-12  nI=0.9507  Rsh=430.0559  Rs=0.43042  BAL=off  Tc=1e-6  Tfilter=5e-5
      settings: SourceProductName=Simscape Electrical
  Suhu : Constant  Value=[25 25 25 25]
  powergui : powerlib/powergui  Priority=1  SimulationMode=Continuous  SampleTime=50e-6  frequency=60  Iterations=50  frequencyindice=0  Pbase=100e6  ErrMax=1e-4  UnitsV=kV  UnitsW=MW  buscounter=0  FunctionMessages=off  echomessages=off  EnableUseOfTLC=off  CurrentSourceSwitches=off  DisableSnubberDevices=off  DisableRonSwitches=off  DisableVfSwitches=off  DisplayEquations=off  AutomaticDiscreteSolvers=off  SolverType=Tustin/Backward Euler (TBE)  Interpol=off  ExternalGateDelay=off  methode=off  Ts=100  x0status=blocks  SPID=on  SwTol=0  HookPort=off  NonlinearTolerance=1e-4  nMaxIteration=100  ContinueOnMaxIteration=off  RestoreLinks=warning  ResistiveCurrentMeasurement=off  Frange=[0:2:500]  Ylog=off  Xlog=on  ShowGrid=off  save=off  variable=ZData  structure=0  ZoomFFT=off  StartTime=0.0  cycles=1  DisplayStyle=1  fundamental=60  FreqAxis=off  MaxFrequency=1000  frequencyindicesteady=1  RmsSteady=1  display=off
      settings: SourceProductName=Simscape Electrical
  Connection Port2 : PMIOPort  Side=Right
  Connection Port3 : PMIOPort  Port=2  Side=Right
  wires:
  Demux3/2 -> PV Module 1/2
  Suhu/1 -> Demux3/1
  Demux2/2 -> PV Module 1/1
  Intensitas Radiasi1/1 -> Demux2/1
  Demux2/3 -> PV Module 2/1
  Demux2/4 -> PV Module 3/1
  Demux3/3 -> PV Module 2/2
  Demux3/1 -> PV Module 5/2
  Demux3/4 -> PV Module 3/2
  Demux2/1 -> PV Module 5/1
  connections:
  Bypass Diode 8/RConn1 -- PV Module 2/RConn2 -- PV Module 3/RConn1 -- Bypass Diode 7/LConn1
  Bypass Diode 8/LConn1 -- PV Module 3/RConn2 -- Connection Port3/RConn1
  Bypass Diode 6/LConn1 -- PV Module 2/RConn1 -- PV Module 1/RConn2 -- Bypass Diode 7/RConn1
  Bypass Diode 5/RConn1 -- PV Module 5/RConn1 -- Connection Port2/RConn1
  PV Module 5/RConn2 -- PV Module 1/RConn1 -- Bypass Diode 5/LConn1 -- Bypass Diode 6/RConn1

== system PSO_BON/Free-Parameter PSO/Panel Surya2 ==
  Diode1 : powerlib/Power Electronics/Diode  Ron=0.001  Lon=0  Vf=0.7  IC=0  UseSnubber=off  Rs=1e5*inf  Cs=inf  Measurements=off
      settings: SourceProductName=Simscape Electrical
  Subsystem : Subsystem  Commented=on
  Subsystem1 : Subsystem  Commented=on
  Subsystem10 : Subsystem
  Subsystem11 : Subsystem
  Subsystem2 : Subsystem  Commented=on
  Subsystem3 : Subsystem  Commented=on
  Subsystem4 : Subsystem
  Subsystem5 : Subsystem
  Subsystem6 : Subsystem
  Subsystem7 : Subsystem
  Subsystem8 : Subsystem
  Subsystem9 : Subsystem
  Temp C{,4..10} (8 alike) : Constant  Value=25
  Connection Port2 : PMIOPort  Side=Right
  Connection Port3 : PMIOPort  Port=2  Side=Right
  wires:
  Subsystem11/1(Out1) -> Subsystem7/1(In1)
  Subsystem8/1(Out1) -> Subsystem4/1(In1)
  Subsystem10/1(Out1) -> Subsystem6/1(In1)
  Subsystem9/1(Out1) -> Subsystem5/1(In1)
  Temp C6/1 -> Subsystem3/2(In2)
  Temp C/1 -> Subsystem/2(In2)
  Temp C5/1 -> Subsystem2/2(In2)
  Temp C4/1 -> Subsystem1/2(In2)
  Temp C7/1 -> Subsystem4/2(In2)
  Temp C8/1 -> Subsystem5/2(In2)
  Temp C9/1 -> Subsystem6/2(In2)
  Temp C10/1 -> Subsystem7/2(In2)
  connections:
  Subsystem7/RConn2 -- Connection Port3/RConn1
  Subsystem4/RConn1 -- Diode1/LConn1
  Subsystem4/RConn2 -- Subsystem5/RConn1
  Subsystem/RConn2 -- Subsystem1/RConn1
  Subsystem2/RConn2 -- Subsystem3/RConn1
  Subsystem1/RConn2 -- Subsystem2/RConn1
  Subsystem6/RConn2 -- Subsystem7/RConn1
  Subsystem5/RConn2 -- Subsystem6/RConn1
  Connection Port2/RConn1 -- Diode1/RConn1

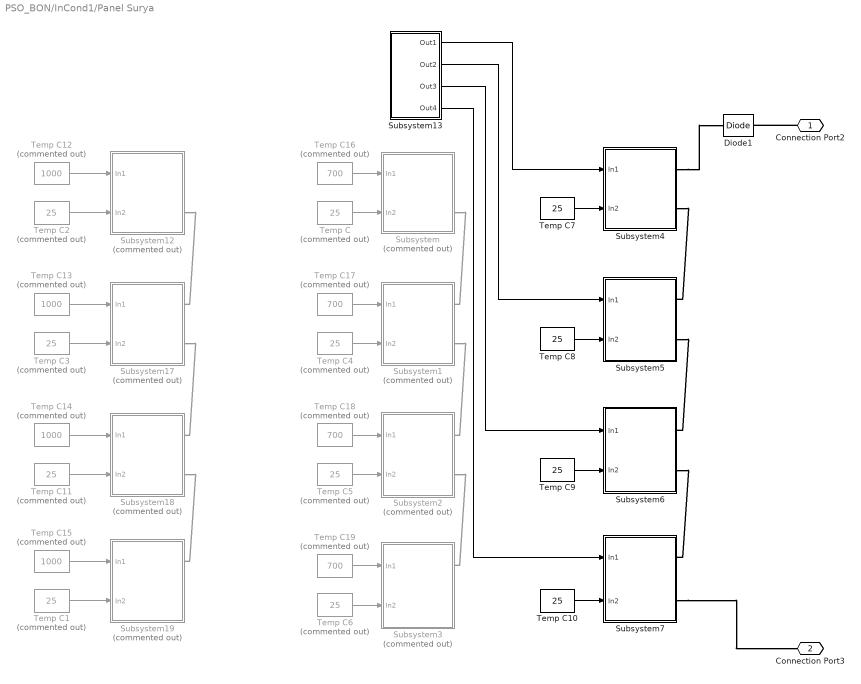
== system PSO_BON/InCond1/Panel Surya ==
  Diode1 : powerlib/Power Electronics/Diode  Ron=0.001  Lon=0  Vf=0.7  IC=0  UseSnubber=off  Rs=1e5*inf  Cs=inf  Measurements=off
      settings: SourceProductName=Simscape Electrical
  Subsystem : Subsystem  Commented=on
  Subsystem1 : Subsystem  Commented=on
  Subsystem12 : Subsystem  Commented=on
  Subsystem13 : Subsystem
  Subsystem17 : Subsystem  Commented=on
  Subsystem18 : Subsystem  Commented=on
  Subsystem19 : Subsystem  Commented=on
  Subsystem2 : Subsystem  Commented=on
  Subsystem3 : Subsystem  Commented=on
  Subsystem4 : Subsystem
  Subsystem5 : Subsystem
  Subsystem6 : Subsystem
  Subsystem7 : Subsystem
  Temp C{,1..6,11} (8 alike) : Constant  Commented=on  Value=25
  Temp C{7..10} (4 alike) : Constant  Value=25
  Temp C{12..15} (4 alike) : Constant  Commented=on  Value=1000
  Temp C{16..19} (4 alike) : Constant  Commented=on  Value=700
  Connection Port2 : PMIOPort  Side=Right
  Connection Port3 : PMIOPort  Port=2  Side=Right
  wires:
  Temp C10/1 -> Subsystem7/2(In2)
  Temp C9/1 -> Subsystem6/2(In2)
  Temp C8/1 -> Subsystem5/2(In2)
  Temp C7/1 -> Subsystem4/2(In2)
  Temp C4/1 -> Subsystem1/2(In2)
  Temp C5/1 -> Subsystem2/2(In2)
  Temp C/1 -> Subsystem/2(In2)
  Temp C6/1 -> Subsystem3/2(In2)
  Subsystem13/2(Out2) -> Subsystem5/1(In1)
  Subsystem13/3(Out3) -> Subsystem6/1(In1)
  Subsystem13/1(Out1) -> Subsystem4/1(In1)
  Subsystem13/4(Out4) -> Subsystem7/1(In1)
  Temp C12/1 -> Subsystem12/1(In1)
  Temp C2/1 -> Subsystem12/2(In2)
  Temp C13/1 -> Subsystem17/1(In1)
  Temp C3/1 -> Subsystem17/2(In2)
  Temp C14/1 -> Subsystem18/1(In1)
  Temp C11/1 -> Subsystem18/2(In2)
  Temp C15/1 -> Subsystem19/1(In1)
  Temp C1/1 -> Subsystem19/2(In2)
  Temp C16/1 -> Subsystem/1(In1)
  Temp C17/1 -> Subsystem1/1(In1)
  Temp C18/1 -> Subsystem2/1(In1)
  Temp C19/1 -> Subsystem3/1(In1)
  connections:
  Connection Port2/RConn1 -- Diode1/RConn1
  Subsystem5/RConn2 -- Subsystem6/RConn1
  Subsystem6/RConn2 -- Subsystem7/RConn1
  Subsystem1/RConn2 -- Subsystem2/RConn1
  Subsystem2/RConn2 -- Subsystem3/RConn1
  Subsystem/RConn2 -- Subsystem1/RConn1
  Subsystem4/RConn2 -- Subsystem5/RConn1
  Subsystem12/RConn2 -- Subsystem17/RConn1
  Subsystem17/RConn2 -- Subsystem18/RConn1
  Subsystem18/RConn2 -- Subsystem19/RConn1
  Subsystem7/RConn2 -- Connection Port3/RConn1
  Subsystem4/RConn1 -- Diode1/LConn1

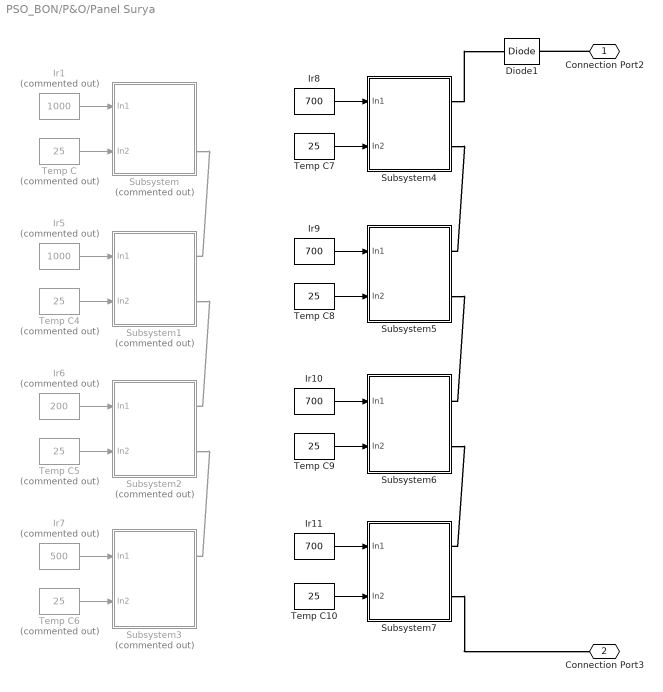
== system PSO_BON/P&O/Panel Surya ==
  Diode1 : powerlib/Power Electronics/Diode  Ron=0.001  Lon=0  Vf=0.7  IC=0  UseSnubber=off  Rs=1e5*inf  Cs=inf  Measurements=off
      settings: SourceProductName=Simscape Electrical
  Ir1 : Constant  Commented=on  Value=1000
  Ir{8..11} (4 alike) : Constant  Value=700
  Ir5 : Constant  Commented=on  Value=1000
  Ir6 : Constant  Commented=on  Value=200
  Ir7 : Constant  Commented=on  Value=500
  Subsystem : Subsystem  Commented=on
  Subsystem1 : Subsystem  Commented=on
  Subsystem2 : Subsystem  Commented=on
  Subsystem3 : Subsystem  Commented=on
  Subsystem4 : Subsystem
  Subsystem5 : Subsystem
  Subsystem6 : Subsystem
  Subsystem7 : Subsystem
  Temp C{,4..6} (4 alike) : Constant  Commented=on  Value=25
  Temp C{7..10} (4 alike) : Constant  Value=25
  Connection Port2 : PMIOPort  Side=Right
  Connection Port3 : PMIOPort  Port=2  Side=Right
  wires:
  Ir7/1 -> Subsystem3/1(In1)
  Temp C6/1 -> Subsystem3/2(In2)
  Ir1/1 -> Subsystem/1(In1)
  Temp C/1 -> Subsystem/2(In2)
  Temp C5/1 -> Subsystem2/2(In2)
  Temp C4/1 -> Subsystem1/2(In2)
  Ir5/1 -> Subsystem1/1(In1)
  Ir6/1 -> Subsystem2/1(In1)
  Ir8/1 -> Subsystem4/1(In1)
  Temp C7/1 -> Subsystem4/2(In2)
  Temp C8/1 -> Subsystem5/2(In2)
  Ir11/1 -> Subsystem7/1(In1)
  Ir9/1 -> Subsystem5/1(In1)
  Temp C9/1 -> Subsystem6/2(In2)
  Ir10/1 -> Subsystem6/1(In1)
  Temp C10/1 -> Subsystem7/2(In2)
  connections:
  Subsystem4/RConn1 -- Diode1/LConn1
  Subsystem7/RConn2 -- Connection Port3/RConn1
  Subsystem4/RConn2 -- Subsystem5/RConn1
  Subsystem/RConn2 -- Subsystem1/RConn1
  Subsystem2/RConn2 -- Subsystem3/RConn1
  Subsystem1/RConn2 -- Subsystem2/RConn1
  Subsystem6/RConn2 -- Subsystem7/RConn1
  Subsystem5/RConn2 -- Subsystem6/RConn1
  Connection Port2/RConn1 -- Diode1/RConn1

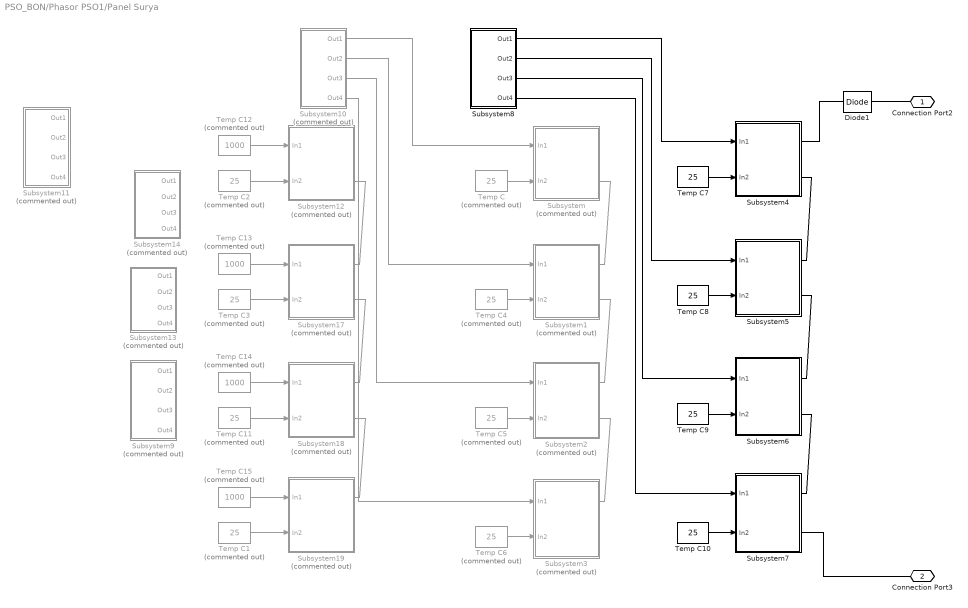
== system PSO_BON/Phasor PSO1/Panel Surya ==
  Diode1 : powerlib/Power Electronics/Diode  Ron=0.001  Lon=0  Vf=0.7  IC=0  UseSnubber=off  Rs=1e5*inf  Cs=inf  Measurements=off
      settings: SourceProductName=Simscape Electrical
  Subsystem : Subsystem  Commented=on
  Subsystem1 : Subsystem  Commented=on
  Subsystem10 : Subsystem  Commented=on
  Subsystem11 : Subsystem  Commented=on
  Subsystem12 : Subsystem  Commented=on
  Subsystem13 : Subsystem  Commented=on
  Subsystem14 : Subsystem  Commented=on
  Subsystem17 : Subsystem  Commented=on
  Subsystem18 : Subsystem  Commented=on
  Subsystem19 : Subsystem  Commented=on
  Subsystem2 : Subsystem  Commented=on
  Subsystem3 : Subsystem  Commented=on
  Subsystem4 : Subsystem
  Subsystem5 : Subsystem
  Subsystem6 : Subsystem
  Subsystem7 : Subsystem
  Subsystem8 : Subsystem
  Subsystem9 : Subsystem  Commented=on
  Temp C{,1..6,11} (8 alike) : Constant  Commented=on  Value=25
  Temp C{7..10} (4 alike) : Constant  Value=25
  Temp C{12..15} (4 alike) : Constant  Commented=on  Value=1000
  Connection Port2 : PMIOPort  Side=Right
  Connection Port3 : PMIOPort  Port=2  Side=Right
  wires:
  Temp C10/1 -> Subsystem7/2(In2)
  Temp C9/1 -> Subsystem6/2(In2)
  Temp C8/1 -> Subsystem5/2(In2)
  Temp C7/1 -> Subsystem4/2(In2)
  Temp C4/1 -> Subsystem1/2(In2)
  Temp C5/1 -> Subsystem2/2(In2)
  Temp C/1 -> Subsystem/2(In2)
  Temp C6/1 -> Subsystem3/2(In2)
  Subsystem8/2(Out2) -> Subsystem5/1(In1)
  Subsystem8/3(Out3) -> Subsystem6/1(In1)
  Subsystem8/1(Out1) -> Subsystem4/1(In1)
  Subsystem8/4(Out4) -> Subsystem7/1(In1)
  Temp C12/1 -> Subsystem12/1(In1)
  Temp C2/1 -> Subsystem12/2(In2)
  Temp C13/1 -> Subsystem17/1(In1)
  Temp C3/1 -> Subsystem17/2(In2)
  Temp C14/1 -> Subsystem18/1(In1)
  Temp C11/1 -> Subsystem18/2(In2)
  Temp C15/1 -> Subsystem19/1(In1)
  Temp C1/1 -> Subsystem19/2(In2)
  Subsystem10/1(Out1) -> Subsystem/1(In1)
  Subsystem10/2(Out2) -> Subsystem1/1(In1)
  Subsystem10/3(Out3) -> Subsystem2/1(In1)
  Subsystem10/4(Out4) -> Subsystem3/1(In1)
  connections:
  Connection Port2/RConn1 -- Diode1/RConn1
  Subsystem5/RConn2 -- Subsystem6/RConn1
  Subsystem6/RConn2 -- Subsystem7/RConn1
  Subsystem1/RConn2 -- Subsystem2/RConn1
  Subsystem2/RConn2 -- Subsystem3/RConn1
  Subsystem/RConn2 -- Subsystem1/RConn1
  Subsystem4/RConn2 -- Subsystem5/RConn1
  Subsystem12/RConn2 -- Subsystem17/RConn1
  Subsystem17/RConn2 -- Subsystem18/RConn1
  Subsystem18/RConn2 -- Subsystem19/RConn1
  Subsystem7/RConn2 -- Connection Port3/RConn1
  Subsystem4/RConn1 -- Diode1/LConn1

== system PSO_BON/Phasor PSO1/Panel Surya1 ==
  Bypass Diode {5..8} (4 alike) : powerlib/Power Electronics/Diode  Ron=0.001  Lon=0  Vf=0.8  IC=0  UseSnubber=off  Rs=500  Cs=250e-9  Measurements=off
      settings: SourceProductName=Simscape Electrical
  Demux2 : Demux
  Demux3 : Demux
  Intensitas Radiasi1 : Constant  Value=[1000 700 100 200]
  PV Module 1 : re_lib/Solar/PV Array  Npar=2  Nser=1  PlotType=array @ 1000 W/m2 & specified temperatures  S_vec="[ 1000  500  100 ]"  Temp_C_vec="[ 45 25  ]"  ModuleName=SunPower SPR-315E-WHT-D  PlotWhenSelected=off  Pm=315.072  Ncell=96  Voc=64.6  Isc=6.14  Vm=54.7  Im=5.76  beta_Voc_pc=-0.27269  alpha_Isc_pc=0.061694  beta_Voc=-0.17616  alpha_Isc=0.003788  IL=6.1461  I0=6.5043e-12  nI=0.9507  Rsh=430.0559  Rs=0.43042  BAL=off  Tc=1e-6  Tfilter=5e-5
      settings: SourceProductName=Simscape Electrical
  PV Module 2 : re_lib/Solar/PV Array  Npar=2  Nser=1  PlotType=array @ 1000 W/m2 & specified temperatures  S_vec="[ 1000  500  100 ]"  Temp_C_vec="[ 45 25  ]"  ModuleName=SunPower SPR-315E-WHT-D  PlotWhenSelected=off  Pm=315.072  Ncell=96  Voc=64.6  Isc=6.14  Vm=54.7  Im=5.76  beta_Voc_pc=-0.27269  alpha_Isc_pc=0.061694  beta_Voc=-0.17616  alpha_Isc=0.003788  IL=6.1461  I0=6.5043e-12  nI=0.9507  Rsh=430.0559  Rs=0.43042  BAL=off  Tc=1e-6  Tfilter=5e-5
      settings: SourceProductName=Simscape Electrical
  PV Module 3 : re_lib/Solar/PV Array  Npar=2  Nser=1  PlotType=array @ 1000 W/m2 & specified temperatures  S_vec="[ 1000  500  100 ]"  Temp_C_vec="[ 45 25  ]"  ModuleName=SunPower SPR-315E-WHT-D  PlotWhenSelected=off  Pm=315.072  Ncell=96  Voc=64.6  Isc=6.14  Vm=54.7  Im=5.76  beta_Voc_pc=-0.27269  alpha_Isc_pc=0.061694  beta_Voc=-0.17616  alpha_Isc=0.003788  IL=6.1461  I0=6.5043e-12  nI=0.9507  Rsh=430.0559  Rs=0.43042  BAL=off  Tc=1e-6  Tfilter=5e-5
      settings: SourceProductName=Simscape Electrical
  PV Module 5 : re_lib/Solar/PV Array  Npar=2  Nser=1  PlotType=one module @ 25 deg.C & specified irradiances  S_vec="[ 1000  800  100 200]"  Temp_C_vec="[ 45 25  ]"  ModuleName=SunPower SPR-315E-WHT-D  PlotWhenSelected=off  Pm=315.072  Ncell=96  Voc=64.6  Isc=6.14  Vm=54.7  Im=5.76  beta_Voc_pc=-0.27269  alpha_Isc_pc=0.061694  beta_Voc=-0.17616  alpha_Isc=0.003788  IL=6.1461  I0=6.5043e-12  nI=0.9507  Rsh=430.0559  Rs=0.43042  BAL=off  Tc=1e-6  Tfilter=5e-5
      settings: SourceProductName=Simscape Electrical
  Suhu : Constant  Value=[25 25 25 25]
  powergui : powerlib/powergui  Priority=1  SimulationMode=Continuous  SampleTime=50e-6  frequency=60  Iterations=50  frequencyindice=0  Pbase=100e6  ErrMax=1e-4  UnitsV=kV  UnitsW=MW  buscounter=0  FunctionMessages=off  echomessages=off  EnableUseOfTLC=off  CurrentSourceSwitches=off  DisableSnubberDevices=off  DisableRonSwitches=off  DisableVfSwitches=off  DisplayEquations=off  AutomaticDiscreteSolvers=off  SolverType=Tustin/Backward Euler (TBE)  Interpol=off  ExternalGateDelay=off  methode=off  Ts=100  x0status=blocks  SPID=on  SwTol=0  HookPort=off  NonlinearTolerance=1e-4  nMaxIteration=100  ContinueOnMaxIteration=off  RestoreLinks=warning  ResistiveCurrentMeasurement=off  Frange=[0:2:500]  Ylog=off  Xlog=on  ShowGrid=off  save=off  variable=ZData  structure=0  ZoomFFT=off  StartTime=0.0  cycles=1  DisplayStyle=1  fundamental=60  FreqAxis=off  MaxFrequency=1000  frequencyindicesteady=1  RmsSteady=1  display=off
      settings: SourceProductName=Simscape Electrical
  Connection Port2 : PMIOPort  Side=Right
  Connection Port3 : PMIOPort  Port=2  Side=Right
  wires:
  Demux2/1 -> PV Module 5/1
  Demux3/4 -> PV Module 3/2
  Demux3/1 -> PV Module 5/2
  Demux3/3 -> PV Module 2/2
  Demux2/4 -> PV Module 3/1
  Demux2/3 -> PV Module 2/1
  Intensitas Radiasi1/1 -> Demux2/1
  Demux2/2 -> PV Module 1/1
  Suhu/1 -> Demux3/1
  Demux3/2 -> PV Module 1/2
  connections:
  Bypass Diode 6/RConn1 -- Bypass Diode 5/LConn1 -- PV Module 1/RConn1 -- PV Module 5/RConn2
  Connection Port2/RConn1 -- PV Module 5/RConn1 -- Bypass Diode 5/RConn1
  Bypass Diode 7/RConn1 -- PV Module 1/RConn2 -- PV Module 2/RConn1 -- Bypass Diode 6/LConn1
  Connection Port3/RConn1 -- PV Module 3/RConn2 -- Bypass Diode 8/LConn1
  Bypass Diode 7/LConn1 -- PV Module 3/RConn1 -- PV Module 2/RConn2 -- Bypass Diode 8/RConn1

== system PSO_BON/Phasor PSO1/Panel Surya2 ==
  Diode1 : powerlib/Power Electronics/Diode  Ron=0.001  Lon=0  Vf=0.7  IC=0  UseSnubber=off  Rs=1e5*inf  Cs=inf  Measurements=off
      settings: SourceProductName=Simscape Electrical
  Subsystem : Subsystem  Commented=on
  Subsystem1 : Subsystem  Commented=on
  Subsystem10 : Subsystem
  Subsystem11 : Subsystem
  Subsystem2 : Subsystem  Commented=on
  Subsystem3 : Subsystem  Commented=on
  Subsystem4 : Subsystem
  Subsystem5 : Subsystem
  Subsystem6 : Subsystem
  Subsystem7 : Subsystem
  Subsystem8 : Subsystem
  Subsystem9 : Subsystem
  Temp C{,4..10} (8 alike) : Constant  Value=25
  Connection Port2 : PMIOPort  Side=Right
  Connection Port3 : PMIOPort  Port=2  Side=Right
  wires:
  Temp C10/1 -> Subsystem7/2(In2)
  Temp C9/1 -> Subsystem6/2(In2)
  Temp C8/1 -> Subsystem5/2(In2)
  Temp C7/1 -> Subsystem4/2(In2)
  Temp C4/1 -> Subsystem1/2(In2)
  Temp C5/1 -> Subsystem2/2(In2)
  Temp C/1 -> Subsystem/2(In2)
  Temp C6/1 -> Subsystem3/2(In2)
  Subsystem9/1(Out1) -> Subsystem5/1(In1)
  Subsystem10/1(Out1) -> Subsystem6/1(In1)
  Subsystem8/1(Out1) -> Subsystem4/1(In1)
  Subsystem11/1(Out1) -> Subsystem7/1(In1)
  connections:
  Connection Port2/RConn1 -- Diode1/RConn1
  Subsystem5/RConn2 -- Subsystem6/RConn1
  Subsystem6/RConn2 -- Subsystem7/RConn1
  Subsystem1/RConn2 -- Subsystem2/RConn1
  Subsystem2/RConn2 -- Subsystem3/RConn1
  Subsystem/RConn2 -- Subsystem1/RConn1
  Subsystem4/RConn2 -- Subsystem5/RConn1
  Subsystem4/RConn1 -- Diode1/LConn1
  Subsystem7/RConn2 -- Connection Port3/RConn1
